simulink model "AngleTrackingTest"  (R2026b)
settings: Solver=FixedStepDiscrete  StopTime=pllTestCfg.Duration  FixedStep=pllCfg.Ts
PostLoadFcn:
  | addpath(fullfile(fileparts(get_param(bdroot,'FileName')),'..','build_process'));initialize_angle_tracking_test(bdroot);
model workspace (MAT data in the model file):
  pllCfg.Ts = 5e-05
  pllCfg.NaturalFrequency = 40
  pllCfg.Damping = 0.707
  pllCfg.Kp = 355.376960974
  pllCfg.Ki = 63165.468167
  pllCfg.Kaw = 502.654824574
  pllCfg.OmegaMax = 1500
  pllCfg.MinMagnitude = 0.5
  pllCfg.LockError = 0.12
  pllCfg.LockSamples = 100
  pllCfg.Theta0 = 0
  pllCfg.Omega0 = 0
  pllTestCfg.Duration = 0.3
  pllTestCfg.ElectricalSpeed = 200
  pllTestCfg.InitialAngle = 0.4
  pllTestCfg.Magnitude = 1
  pllTestCfg.Enable = 1
  pllTestCfg.Reset = 0
  testStim.time = [0 5e-05 0.0001 0.00015 0.0002 0.00025 0.0003 0.00035 0.0004 0.00045 0.0005 0.00055 ... (6001 elements, 6001x1)]
  testStim.signals.values = [0.4 0.41 0.42 0.43 0.44 0.45 0.46 0.47 0.48 0.49 0.5 0.51 ... (36006 elements, 6001x6)]
  testStim.signals.dimensions = 6
libraries: AngleTracking x1
settings Model: Creator=24322  LastModifiedBy=24322

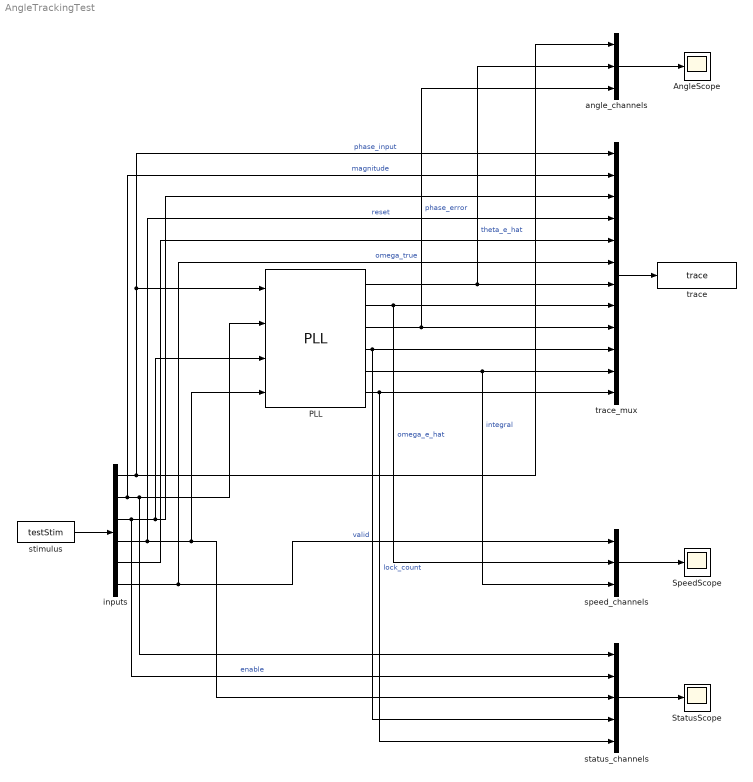
== system AngleTrackingTest ==
  AngleScope : Scope
  PLL : AngleTracking/PLL  pllCfg=pllCfg
  SpeedScope : Scope
  StatusScope : Scope
  angle_channels : Mux  Inputs=3
  inputs : Demux  Outputs=6
  speed_channels : Mux  Inputs=3
  status_channels : Mux  Inputs=5
  stimulus : FromWorkspace  VariableName=testStim  SampleTime=pllCfg.Ts  Interpolate=off  OutputAfterFinalValue=Holding final value
  trace : ToWorkspace  VariableName=trace  SaveFormat=Structure With Time  SampleTime=-1
  trace_mux : Mux  Inputs=12
  wires:
  status_channels/1 -> StatusScope/1
  speed_channels/1 -> SpeedScope/1
  angle_channels/1 -> AngleScope/1
  trace_mux/1 -> trace/1
  PLL/6 -> trace_mux/12, status_channels/5  "lock_count"
  inputs/6 -> trace_mux/6, speed_channels/1  "omega_true"
  PLL/5 -> trace_mux/11, speed_channels/3  "integral"
  inputs/5 -> trace_mux/5
  PLL/4 -> trace_mux/10, status_channels/4  "valid"
  PLL/3 -> trace_mux/9, angle_channels/3  "phase_error"
  PLL/2 -> trace_mux/8, speed_channels/2  "omega_e_hat"
  PLL/1 -> trace_mux/7, angle_channels/2  "theta_e_hat"
  inputs/4 -> PLL/4, status_channels/3, trace_mux/4  "reset"
  inputs/3 -> PLL/3, trace_mux/3, status_channels/2  "enable"
  inputs/2 -> PLL/2, status_channels/1, trace_mux/2  "magnitude"
  inputs/1 -> trace_mux/1, PLL/1, angle_channels/1  "phase_input"
  stimulus/1 -> inputs/1
